simulink model "LQRconlacnguoc"  (R2024b)
settings: Solver=ode45  StartTime=0.0  StopTime=60  FixedStep=0.001  MaxStep=0.01  RelTol=1e-3
values from neighbouring files (symbols this model uses):
  D = [0; 0]    [K_vector_2.m]
libraries: simulink x20, slpidlib x11, slctrl_smc x5, mpclib x1, dspstat3 x1, rllib x1
(part 1 of 3)
settings Model: Creator=DELL  LastModifiedBy=minhh
settings RTWCC: GenCodeOnly=on

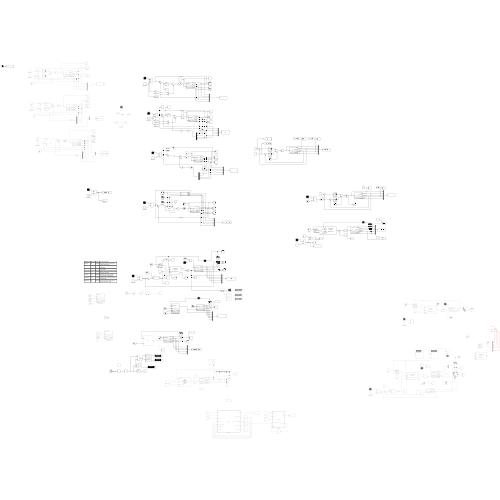
[thumbnail: Simulink's stored preview of the top-level diagram]
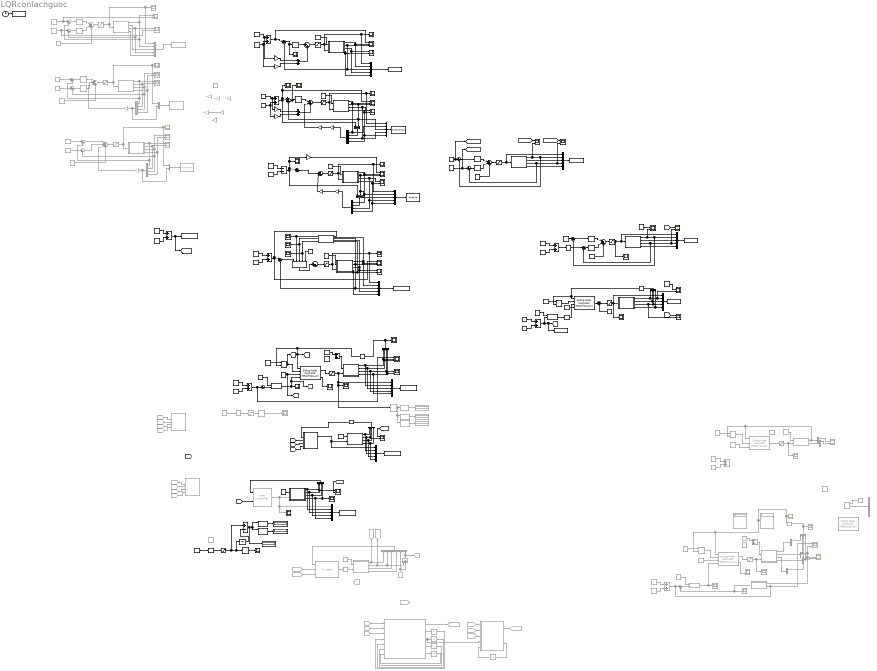
== system LQRconlacnguoc ==
  note: To Improve...
      | Parameter
      | Action
      | The "Physics" Reason
      |
      | Rise Time
      | Eta
      | Increase
      | It increases the force used to "jump" onto the sliding surface.
      |
      | Rise Time
      | C (Slope)
      | Increase
      | It makes the "slide" toward the target much steeper.
      |
      | Settling Time
      | C (Slope)
      | Increase
      | Faster convergence once the system is on the surface.
      |
      | Settling Time
      | Phi
      | Increase
      | Reduces "bouncing" at the target, letting the system rest sooner.
      |
      | S.S. Error
      | Phi
      | Decrease
      | Shrinks the "lazy zone" where the controller stops being aggressive.
      |
      | Smoothness
      | Phi
      | Increase
      | Softens the high-frequency switching (kills chattering).
      |
      | Smoothness
      | Eta
      | Decrease
      | Prevents the system from hitting the sliding surface too violently.
  A : Constant  Commented=on  Value=[0 0 0 0; 0 0 0 1; -4 1 -0.5 0.4; 0.833 -0.833 0.333 -0.333]
  A_1 : Constant  Commented=on  Value=[0, 1; -3, -0.2]
  A_2 : Constant  Commented=on  Value=[0, 0, 0, 0; 0, 0, 0, 1; -4, 1, -0.5, 0.4; 0.833, -0.833, 0.333, -0.333]  VectorParams1D=off
  A_3 : Constant  Value=[0, 0, 0, 0; 0, 0, 0, 1; -4, 1, -0.5, 0.4; 0.833, -0.833, 0.333, -0.333]  VectorParams1D=off
  A_4 : Constant  Value=[0, 1, 0, 0; 29.8310, 0, 0, 0; 0, 0, 0, 1; -0.9392, 0, 0, 0]  VectorParams1D=off
  Add{,2..3,5..7,12..13,16,18} (10 alike) : Sum
  Add1 : Sum  Commented=on
  Add10 : Sum  Commented=on
  Add11 : Sum  Commented=on
  Add14 : Sum  Commented=on  Inputs=-+
  Add15 : Sum  Inputs=+-
  Add4 : Sum  Inputs=+-
  Add8 : Sum  Inputs=--
  Add9 : Sum  Inputs=+-
  Assignment : Assignment  Commented=on  DiagnosticForDimensions=Warning  IndexOptions=Index vector (dialog)  Indices=2  OutputSizes=1
  Assignment1 : Assignment  DiagnosticForDimensions=Warning  IndexOptions=Index vector (dialog)  Indices=2  OutputSizes=1
  Assignment2 : Assignment  DiagnosticForDimensions=Warning  IndexOptions=Index vector (dialog)  Indices=3  OutputSizes=1
  B : Constant  Commented=on  Value=[0; 0.004]
  B1 : Constant  Commented=on  Value=[0; 0; 0.004; 0]
  B2 : Constant  Commented=on  Value=[0; 0.004; 0; 0]
  B3 : Constant  Value=[0; 0.004; 0; 0]
  B4 : Constant  Value=[0; -1.1574; 0; 0.4167]
  Band-Limited White Noise : simulink/Sources/Band-Limited White Noise  Commented=on  Cov=[0.001]  Ts=0.01  seed=[23341]
  Band-Limited White Noise1 : simulink/Sources/Band-Limited White Noise  Commented=on  Cov=[0.001]  Ts=0.01  seed=[23341]
  Band-Limited White Noise{3..5,7,9..11} (7 alike) : simulink/Sources/Band-Limited White Noise  Cov=[200]  Ts=0.01  seed=[23341]
  Band-Limited White Noise12 : simulink/Sources/Band-Limited White Noise  Commented=on  Cov=[200]  Ts=0.01  seed=[23341]
  Band-Limited White Noise13 : simulink/Sources/Band-Limited White Noise  Cov=[0.001]  Ts=0.01  seed=[23341]
  Band-Limited White Noise14 : simulink/Sources/Band-Limited White Noise  Cov=[0.001]  Ts=0.01  seed=[23341]
  Band-Limited White Noise15 : simulink/Sources/Band-Limited White Noise  Cov=[0.001]  Ts=0.01  seed=[23341]
  Band-Limited White Noise2 : simulink/Sources/Band-Limited White Noise  Commented=on  Cov=[0.001]  Ts=0.01  seed=[23341]
  Band-Limited White Noise6 : simulink/Sources/Band-Limited White Noise  Commented=on  Cov=[200]  Ts=0.01  seed=[23341]
  Band-Limited White Noise8 : simulink/Sources/Band-Limited White Noise  Commented=on  Cov=[200]  Ts=0.01  seed=[23341]
  Clock : Clock
      settings: Decimation=100
  Constant : Constant  Commented=on  Value=[0; 0; 0; 0]  VectorParams1D=off
  Constant1 : Constant  Value=[0; 0; 0; 0]  VectorParams1D=off
  Constant2 : Constant  Value=[0; 0; 0; 0]  VectorParams1D=off
  Constant3 : Constant  Value=0
  D_values : Scope
  Demux{,1..5} (6 alike) : Demux  Commented=on  Outputs=2
  Display{,1,5..7} (5 alike) : Display  Commented=on
  Display2 : Display
  Display3 : Display
  Display4 : Display
  Feedforward : Gain  Gain=130  Multiplication=Matrix(K*u)
  Feedforward1 : Gain  Gain=200  Multiplication=Matrix(K*u)
  Feedforward2 : Gain  Gain=300  Multiplication=Matrix(K*u)
  Feedforward3 : Gain  Gain=300  Multiplication=Matrix(K*u)
  From : From  Commented=on  GotoTag=f_x
  From1 : From  Commented=on  GotoTag=x
  From10 : From  Commented=on  GotoTag=x
  From11 : From  Commented=on  GotoTag=g_x
  From12 : From  Commented=on  GotoTag=x_ref
  From15 : From  Commented=on  GotoTag=NN_x2_ref
  From16 : From  Commented=on  GotoTag=NN_Error
  From17 : From  Commented=on  GotoTag=NN_u
  From18 : From  Commented=on  GotoTag=NN_x1
  From19 : From  Commented=on  GotoTag=NN_x2
  From2 : From  Commented=on  GotoTag=g_x
  From20 : From  Commented=on  GotoTag=NN_x2_ref
  From21 : From  Commented=on  GotoTag=NN_x2
  From22 : From  Commented=on  GotoTag=NN_x2_ref
  From23 : From  Commented=on  GotoTag=NN_IsDone
  From24 : From  Commented=on  GotoTag=NN_Reward
  From3 : From  Commented=on  GotoTag=x_ref
  From9 : From  Commented=on  GotoTag=f_x
  Gain1 : Gain  Commented=on  Gain=[-137.7896 -25.9783 -22.3607 -27.5768]  Multiplication=Matrix(K*u)
  Gain10 : Gain  Commented=on  Gain=10000  Multiplication=Matrix(K*u)
  Gain11 : Gain  Commented=on  Gain=[-31.2820 70.3549 95.2844 249.5836]  Multiplication=Matrix(K*u)
  Gain12 : Gain  Commented=on  Gain=[-0.5120 271.0493 500.9119 924.2311]  Multiplication=Matrix(K*u)
  Gain13 : Gain  Gain=-1  Multiplication=Matrix(K*u)
  Gain14 : Gain  Gain="[242.4879  684.9939   85.7051  920.8251]"  Multiplication=Matrix(K*u)
  Gain2 : Gain  Commented=on  Gain=[-137.7896 -25.9783 -22.3607 -27.5768]  Multiplication=Matrix(K*u)
  Gain3 : Gain  Gain="[197.1274  543.9573  131.0655  963.0780]"  Multiplication=Matrix(K*u)
  Gain4 : Gain  Commented=on  Gain=[1.6728 1.0816 0.3095 1.2849]  Multiplication=Matrix(K*u)
  Gain5 : Gain  Commented=on  Gain=[-0.4237 1.7558 1.8822 4.6801]  Multiplication=Matrix(K*u)
  Gain6 : Gain  Multiplication=Matrix(K*u)
  Gain7 : Gain  Gain=.66  Multiplication=Matrix(K*u)
  Gain8 : Gain  Commented=on  Gain=[1.6728 1.0816 0.3095 1.2849]  Multiplication=Matrix(K*u)
  Goto10 : Goto  Commented=on  GotoTag=NN_x2
  Goto5 : Goto  Commented=on  GotoTag=NN_Error
  Goto6 : Goto  Commented=on  GotoTag=NN_u
  Goto7 : Goto  Commented=on  GotoTag=NN_Reward
  Goto8 : Goto  Commented=on  GotoTag=NN_IsDone
  Goto9 : Goto  Commented=on  GotoTag=NN_x1
  I_values : Scope
  IsDone : MATLAB Function  Commented=on  TreatAsAtomicUnit=on
  MPC Controller : mpclib/MPC Controller  Commented=on  SCDEnableBlockLinearizationSpecification=on  mpcobj=mpc1  is_multiple=0  enable_value=0  return_u0=off  updateMPCinCallerWorkspace=on  md_inport=off  mv_inport=off  uref_inport=off  return_cost=off  return_mvseq=off  return_qpstatus=off  return_xseq=off  return_state=off  return_ovseq=off  state_inport=off  umin_inport=off  umax_inport=off  ymin_inport=off  ymax_inport=off  cc_inport=off  ywt_inport=off  uwt_inport=off  duwt_inport=off  rhoeps_inport=off  pm_inport=off  MaximumP=10  HorizonChoice=FixedHorizon  n_ts=0.01  n_p=50  n_mv=1  n_md=0  n_ud=0  n_mo=4  n_uo=0  BlockDataType=double  SampleTimeInherited=off  switch_inport=off
  Manual SMC : Subsystem  Commented=on
  Manual SMC Adaptive : Subsystem
  MatrixMultiply : Product  Commented=on  Multiplication=Matrix(*)
  MatrixMultiply1 : Product  Commented=on  Multiplication=Matrix(*)
  MatrixMultiply2 : Product  Commented=on  Multiplication=Matrix(*)
  MatrixMultiply3 : Product  Multiplication=Matrix(*)
  MatrixMultiply4 : Product  Multiplication=Matrix(*)
  Mean : dspstat3/Mean  Commented=on  run=on  InputProcessing=Columns as channels (frame based)  reset_popup=None  directionMode=Each column  dimension=1  roiEnable=off  roiType=Rectangles  roiPortion=Entire ROI  roiOutput=Individual statistics for each ROI  roiFlag=off  roundingMode=Floor  overflowMode=off  outputDataTypeStr=Inherit: Same as accumulator  outputMin=[]  outputMax=[]  outputLastDataTypeStr=Inherit: Same as accumulator
  MinMax Running Resettable : simulink/Math Operations/MinMax Running Resettable  Function=min  vinit=0.0
  MinMax Running Resettable1 : simulink/Math Operations/MinMax Running Resettable  Function=max  vinit=0.0
  MinMax Running Resettable2 : simulink/Math Operations/MinMax Running Resettable  Commented=on  Function=min  vinit=0.0
  MinMax Running Resettable3 : simulink/Math Operations/MinMax Running Resettable  Commented=on  Function=max  vinit=0.0
  Mux{,1,11,13} (4 alike) : Mux  Commented=on
  Mux{7,9..10,14,16..18,20..22} (10 alike) : Mux  Inputs=5
  Mux{5..6,8,12,15,23} (6 alike) : Mux
  Mux19 : Mux  Commented=on  Inputs=6
  Mux2 : Mux  Commented=on  Inputs=2
  Mux3 : Mux  Commented=on  Inputs=2
  Mux4 : Mux  Commented=on  Inputs=5
  N : Constant  Value=100
  PI : Subsystem  Commented=on
  PID Controller : slpidlib/PID Controller  Commented=on  Controller=PID  Form=Parallel  TimeDomain=Continuous-time  UseExternalTs=off  SampleTime=-1  IntegratorMethod=Forward Euler  FilterMethod=Forward Euler  ControllerParametersSource=internal  P=-40  I=0  UseKiTs=off  D=-8  UseExternalDerivativeSource=off  N=100  UseFilter=on  TunerSelectOption=Transfer Function Based (PID Tuner App)  InitialConditionSource=internal  InitialConditionForIntegrator=0  InitialConditionForFilter=0  DifferentiatorICPrevScaledInput=0  ExternalReset=none  TrackingMode=off  Kt=1  LimitOutput=on  SatLimitsSource=internal  UpperSaturationLimit=1  LowerSaturationLimit=-1  LinearizeAsGain=on  AntiWindupMode=none  Kb=1  LimitIntegrator=off  UpperIntegratorSaturationLimit=inf  LowerIntegratorSaturationLimit=-inf  POutMin=[]  POutMax=[]  IOutMin=[]  IOutMax=[]  DOutMin=[]  DOutMax=[]  NOutMin=[]  NOutMax=[]  SumOutMin=[]  SumOutMax=[]  SaturationOutMin=[]  SaturationOutMax=[]  PParamMin=[]  PParamMax=[]  IParamMin=[]  IParamMax=[]  DParamMin=[]  DParamMax=[]  NParamMin=[]  NParamMax=[]  KbParamMin=[]  KbParamMax=[]  KtParamMin=[]  KtParamMax=[]  KbOutMin=[]  KbOutMax=[]  KtOutMin=[]  KtOutMax=[]  IntegratorOutMin=[]  IntegratorOutMax=[]  FilterOutMin=[]  FilterOutMax=[]  SumI1OutMin=[]  SumI1OutMax=[]  SumI2OutMin=[]  SumI2OutMax=[]  SumI3OutMin=[]  SumI3OutMax=[]  SumI4OutMin=[]  SumI4OutMax=[]  SumDOutMin=[]  SumDOutMax=[]  DifferentiatorOutMin=[]  DifferentiatorOutMax=[]  FilterDiffOutCoefMin=[]  FilterDiffOutCoefMax=[]  ReciprocalOutMin=[]  ReciprocalOutMax=[]  SumDenOutMin=[]  SumDenOutMax=[]  SumNumOutMin=[]  SumNumOutMax=[]  DivideOutMin=[]  DivideOutMax=[]  UdiffTsProdOutMin=[]  UdiffTsProdOutMax=[]  NTsProdOutMin=[]  NTsProdOutMax=[]  UintegralTsProdOutMin=[]  UintegralTsProdOutMax=[]  UngainTsProdOutMin=[]  UngainTsProdOutMax=[]  ClampingZeroOutDataTypeStr=Inherit: Inherit via back propagation  ClampingZeroOutMin=[]  ClampingZeroOutMax=[]  FilterDenConstantOutDataTypeStr=Inherit: Inherit via back propagation  FilterDenConstantOutMin=[]  FilterDenConstantOutMax=[]  PCopyOutDataTypeStr=Inherit: Inherit via back propagation  PCopyOutMin=[]  PCopyOutMax=[]  NCopyOutDataTypeStr=Inherit: Inherit via back propagation  NCopyOutMin=[]  NCopyOutMax=[]  IntegratorContinuousStateAttributes=''  IntegratorStateMustResolveToSignalObject=off  IntegratorRTWStateStorageClass=Auto  FilterContinuousStateAttributes=''  FilterStateMustResolveToSignalObject=off  FilterRTWStateStorageClass=Auto  ParallelPVariant=InternalParameters  IdealPVariant=Disabled  IVariant=InternalParameters  DVariant=InternalParameters  IntegratorVariant=Continuous  SatVariant=Enabled  AWVariant=Passthrough  PCopyVariant=Disabled  TRVariant=Disabled  FdbkBlocksVariant=Forward  IdealPFdbkVariant=Disabled  SatFdbkVariant=Disabled  DerivativeFilterVariant=ContFilter  NVariant=InternalParameters  NCopyVariant=Disabled  FilterICVariant=InternalICsFilter  IntegratorICVariant=InternalICs  ExternalResetVariant=Disabled  TRSumVariant=Passthrough  SumFdbkVariant=Disabled  SumVariant=Sum_PID  TsampFilterVariant=InternalTs  TsampNgainVariant=Passthrough  TsampIntegralVariant=Disabled_SignalSpec  ExternalSaturationOutDataTypeStr=Inherit: Same as second input  DerivativeSourceVariant=ErrorSignal  PreIntVariant=InternalPreInt
  PID Controller1 : slpidlib/PID Controller  Commented=on  Controller=PID  Form=Parallel  TimeDomain=Continuous-time  UseExternalTs=off  SampleTime=-1  IntegratorMethod=Forward Euler  FilterMethod=Forward Euler  ControllerParametersSource=internal  P=-1.25  I=0  UseKiTs=off  D=-3.6  UseExternalDerivativeSource=off  N=100  UseFilter=on  TunerSelectOption=Transfer Function Based (PID Tuner App)  InitialConditionSource=internal  InitialConditionForIntegrator=0  InitialConditionForFilter=0  DifferentiatorICPrevScaledInput=0  ExternalReset=none  TrackingMode=off  Kt=1  LimitOutput=on  SatLimitsSource=internal  UpperSaturationLimit=0.1  LowerSaturationLimit=-0.1  LinearizeAsGain=on  AntiWindupMode=none  Kb=1  LimitIntegrator=off  UpperIntegratorSaturationLimit=inf  LowerIntegratorSaturationLimit=-inf  POutMin=[]  POutMax=[]  IOutMin=[]  IOutMax=[]  DOutMin=[]  DOutMax=[]  NOutMin=[]  NOutMax=[]  SumOutMin=[]  SumOutMax=[]  SaturationOutMin=[]  SaturationOutMax=[]  PParamMin=[]  PParamMax=[]  IParamMin=[]  IParamMax=[]  DParamMin=[]  DParamMax=[]  NParamMin=[]  NParamMax=[]  KbParamMin=[]  KbParamMax=[]  KtParamMin=[]  KtParamMax=[]  KbOutMin=[]  KbOutMax=[]  KtOutMin=[]  KtOutMax=[]  IntegratorOutMin=[]  IntegratorOutMax=[]  FilterOutMin=[]  FilterOutMax=[]  SumI1OutMin=[]  SumI1OutMax=[]  SumI2OutMin=[]  SumI2OutMax=[]  SumI3OutMin=[]  SumI3OutMax=[]  SumI4OutMin=[]  SumI4OutMax=[]  SumDOutMin=[]  SumDOutMax=[]  DifferentiatorOutMin=[]  DifferentiatorOutMax=[]  FilterDiffOutCoefMin=[]  FilterDiffOutCoefMax=[]  ReciprocalOutMin=[]  ReciprocalOutMax=[]  SumDenOutMin=[]  SumDenOutMax=[]  SumNumOutMin=[]  SumNumOutMax=[]  DivideOutMin=[]  DivideOutMax=[]  UdiffTsProdOutMin=[]  UdiffTsProdOutMax=[]  NTsProdOutMin=[]  NTsProdOutMax=[]  UintegralTsProdOutMin=[]  UintegralTsProdOutMax=[]  UngainTsProdOutMin=[]  UngainTsProdOutMax=[]  ClampingZeroOutDataTypeStr=Inherit: Inherit via back propagation  ClampingZeroOutMin=[]  ClampingZeroOutMax=[]  FilterDenConstantOutDataTypeStr=Inherit: Inherit via back propagation  FilterDenConstantOutMin=[]  FilterDenConstantOutMax=[]  PCopyOutDataTypeStr=Inherit: Inherit via back propagation  PCopyOutMin=[]  PCopyOutMax=[]  NCopyOutDataTypeStr=Inherit: Inherit via back propagation  NCopyOutMin=[]  NCopyOutMax=[]  IntegratorContinuousStateAttributes=''  IntegratorStateMustResolveToSignalObject=off  IntegratorRTWStateStorageClass=Auto  FilterContinuousStateAttributes=''  FilterStateMustResolveToSignalObject=off  FilterRTWStateStorageClass=Auto  ParallelPVariant=InternalParameters  IdealPVariant=Disabled  IVariant=InternalParameters  DVariant=InternalParameters  IntegratorVariant=Continuous  SatVariant=Enabled  AWVariant=Passthrough  PCopyVariant=Disabled  TRVariant=Disabled  FdbkBlocksVariant=Forward  IdealPFdbkVariant=Disabled  SatFdbkVariant=Disabled  DerivativeFilterVariant=ContFilter  NVariant=InternalParameters  NCopyVariant=Disabled  FilterICVariant=InternalICsFilter  IntegratorICVariant=InternalICs  ExternalResetVariant=Disabled  TRSumVariant=Passthrough  SumFdbkVariant=Disabled  SumVariant=Sum_PID  TsampFilterVariant=InternalTs  TsampNgainVariant=Passthrough  TsampIntegralVariant=Disabled_SignalSpec  ExternalSaturationOutDataTypeStr=Inherit: Same as second input  DerivativeSourceVariant=ErrorSignal  PreIntVariant=InternalPreInt
  PID Controller2 : slpidlib/PID Controller  Commented=on  Controller=PID  Form=Parallel  TimeDomain=Continuous-time  UseExternalTs=off  SampleTime=-1  IntegratorMethod=Forward Euler  FilterMethod=Forward Euler  ControllerParametersSource=internal  P=1  I=1  UseKiTs=off  D=1  UseExternalDerivativeSource=off  N=100  UseFilter=on  TunerSelectOption=Transfer Function Based (PID Tuner App)  InitialConditionSource=internal  InitialConditionForIntegrator=0  InitialConditionForFilter=0  DifferentiatorICPrevScaledInput=0  ExternalReset=none  TrackingMode=off  Kt=1  LimitOutput=off  SatLimitsSource=internal  UpperSaturationLimit=1  LowerSaturationLimit=-1  LinearizeAsGain=on  AntiWindupMode=none  Kb=1  LimitIntegrator=off  UpperIntegratorSaturationLimit=inf  LowerIntegratorSaturationLimit=-inf  POutMin=[]  POutMax=[]  IOutMin=[]  IOutMax=[]  DOutMin=[]  DOutMax=[]  NOutMin=[]  NOutMax=[]  SumOutMin=[]  SumOutMax=[]  SaturationOutMin=[]  SaturationOutMax=[]  PParamMin=[]  PParamMax=[]  IParamMin=[]  IParamMax=[]  DParamMin=[]  DParamMax=[]  NParamMin=[]  NParamMax=[]  KbParamMin=[]  KbParamMax=[]  KtParamMin=[]  KtParamMax=[]  KbOutMin=[]  KbOutMax=[]  KtOutMin=[]  KtOutMax=[]  IntegratorOutMin=[]  IntegratorOutMax=[]  FilterOutMin=[]  FilterOutMax=[]  SumI1OutMin=[]  SumI1OutMax=[]  SumI2OutMin=[]  SumI2OutMax=[]  SumI3OutMin=[]  SumI3OutMax=[]  SumI4OutMin=[]  SumI4OutMax=[]  SumDOutMin=[]  SumDOutMax=[]  DifferentiatorOutMin=[]  DifferentiatorOutMax=[]  FilterDiffOutCoefMin=[]  FilterDiffOutCoefMax=[]  ReciprocalOutMin=[]  ReciprocalOutMax=[]  SumDenOutMin=[]  SumDenOutMax=[]  SumNumOutMin=[]  SumNumOutMax=[]  DivideOutMin=[]  DivideOutMax=[]  UdiffTsProdOutMin=[]  UdiffTsProdOutMax=[]  NTsProdOutMin=[]  NTsProdOutMax=[]  UintegralTsProdOutMin=[]  UintegralTsProdOutMax=[]  UngainTsProdOutMin=[]  UngainTsProdOutMax=[]  ClampingZeroOutDataTypeStr=Inherit: Inherit via back propagation  ClampingZeroOutMin=[]  ClampingZeroOutMax=[]  FilterDenConstantOutDataTypeStr=Inherit: Inherit via back propagation  FilterDenConstantOutMin=[]  FilterDenConstantOutMax=[]  PCopyOutDataTypeStr=Inherit: Inherit via back propagation  PCopyOutMin=[]  PCopyOutMax=[]  NCopyOutDataTypeStr=Inherit: Inherit via back propagation  NCopyOutMin=[]  NCopyOutMax=[]  IntegratorContinuousStateAttributes=''  IntegratorStateMustResolveToSignalObject=off  IntegratorRTWStateStorageClass=Auto  FilterContinuousStateAttributes=''  FilterStateMustResolveToSignalObject=off  FilterRTWStateStorageClass=Auto  ParallelPVariant=InternalParameters  IdealPVariant=Disabled  IVariant=InternalParameters  DVariant=InternalParameters  IntegratorVariant=Continuous  SatVariant=Disabled  AWVariant=Passthrough  PCopyVariant=Disabled  TRVariant=Disabled  FdbkBlocksVariant=Forward  IdealPFdbkVariant=Disabled  SatFdbkVariant=Disabled  DerivativeFilterVariant=ContFilter  NVariant=InternalParameters  NCopyVariant=Disabled  FilterICVariant=InternalICsFilter  IntegratorICVariant=InternalICs  ExternalResetVariant=Disabled  TRSumVariant=Passthrough  SumFdbkVariant=Disabled  SumVariant=Sum_PID  TsampFilterVariant=InternalTs  TsampNgainVariant=Passthrough  TsampIntegralVariant=Disabled_SignalSpec  ExternalSaturationOutDataTypeStr=Inherit: Same as second input  DerivativeSourceVariant=ErrorSignal  PreIntVariant=InternalPreInt
  PID Controller3 : slpidlib/PID Controller  Commented=on  Controller=PID  Form=Parallel  TimeDomain=Continuous-time  UseExternalTs=off  SampleTime=-1  IntegratorMethod=Forward Euler  FilterMethod=Forward Euler  ControllerParametersSource=internal  P=1.5  I=-7.5  UseKiTs=off  D=5  UseExternalDerivativeSource=off  N=100  UseFilter=on  TunerSelectOption=Transfer Function Based (PID Tuner App)  InitialConditionSource=internal  InitialConditionForIntegrator=0  InitialConditionForFilter=0  DifferentiatorICPrevScaledInput=0  ExternalReset=none  TrackingMode=off  Kt=1  LimitOutput=off  SatLimitsSource=internal  UpperSaturationLimit=0.1  LowerSaturationLimit=-0.1  LinearizeAsGain=on  AntiWindupMode=none  Kb=1  LimitIntegrator=off  UpperIntegratorSaturationLimit=inf  LowerIntegratorSaturationLimit=-inf  POutMin=[]  POutMax=[]  IOutMin=[]  IOutMax=[]  DOutMin=[]  DOutMax=[]  NOutMin=[]  NOutMax=[]  SumOutMin=[]  SumOutMax=[]  SaturationOutMin=[]  SaturationOutMax=[]  PParamMin=[]  PParamMax=[]  IParamMin=[]  IParamMax=[]  DParamMin=[]  DParamMax=[]  NParamMin=[]  NParamMax=[]  KbParamMin=[]  KbParamMax=[]  KtParamMin=[]  KtParamMax=[]  KbOutMin=[]  KbOutMax=[]  KtOutMin=[]  KtOutMax=[]  IntegratorOutMin=[]  IntegratorOutMax=[]  FilterOutMin=[]  FilterOutMax=[]  SumI1OutMin=[]  SumI1OutMax=[]  SumI2OutMin=[]  SumI2OutMax=[]  SumI3OutMin=[]  SumI3OutMax=[]  SumI4OutMin=[]  SumI4OutMax=[]  SumDOutMin=[]  SumDOutMax=[]  DifferentiatorOutMin=[]  DifferentiatorOutMax=[]  FilterDiffOutCoefMin=[]  FilterDiffOutCoefMax=[]  ReciprocalOutMin=[]  ReciprocalOutMax=[]  SumDenOutMin=[]  SumDenOutMax=[]  SumNumOutMin=[]  SumNumOutMax=[]  DivideOutMin=[]  DivideOutMax=[]  UdiffTsProdOutMin=[]  UdiffTsProdOutMax=[]  NTsProdOutMin=[]  NTsProdOutMax=[]  UintegralTsProdOutMin=[]  UintegralTsProdOutMax=[]  UngainTsProdOutMin=[]  UngainTsProdOutMax=[]  ClampingZeroOutDataTypeStr=Inherit: Inherit via back propagation  ClampingZeroOutMin=[]  ClampingZeroOutMax=[]  FilterDenConstantOutDataTypeStr=Inherit: Inherit via back propagation  FilterDenConstantOutMin=[]  FilterDenConstantOutMax=[]  PCopyOutDataTypeStr=Inherit: Inherit via back propagation  PCopyOutMin=[]  PCopyOutMax=[]  NCopyOutDataTypeStr=Inherit: Inherit via back propagation  NCopyOutMin=[]  NCopyOutMax=[]  IntegratorContinuousStateAttributes=''  IntegratorStateMustResolveToSignalObject=off  IntegratorRTWStateStorageClass=Auto  FilterContinuousStateAttributes=''  FilterStateMustResolveToSignalObject=off  FilterRTWStateStorageClass=Auto  ParallelPVariant=InternalParameters  IdealPVariant=Disabled  IVariant=InternalParameters  DVariant=InternalParameters  IntegratorVariant=Continuous  SatVariant=Disabled  AWVariant=Passthrough  PCopyVariant=Disabled  TRVariant=Disabled  FdbkBlocksVariant=Forward  IdealPFdbkVariant=Disabled  SatFdbkVariant=Disabled  DerivativeFilterVariant=ContFilter  NVariant=InternalParameters  NCopyVariant=Disabled  FilterICVariant=InternalICsFilter  IntegratorICVariant=InternalICs  ExternalResetVariant=Disabled  TRSumVariant=Passthrough  SumFdbkVariant=Disabled  SumVariant=Sum_PID  TsampFilterVariant=InternalTs  TsampNgainVariant=Passthrough  TsampIntegralVariant=Disabled_SignalSpec  ExternalSaturationOutDataTypeStr=Inherit: Same as second input  DerivativeSourceVariant=ErrorSignal  PreIntVariant=InternalPreInt
  PID Controller4 : slpidlib/PID Controller  Controller=PID  Form=Parallel  TimeDomain=Continuous-time  UseExternalTs=off  SampleTime=-1  IntegratorMethod=Forward Euler  FilterMethod=Forward Euler  ControllerParametersSource=internal  P=12000  I=1100  UseKiTs=off  D=5000  UseExternalDerivativeSource=off  N=100  UseFilter=on  TunerSelectOption=Transfer Function Based (PID Tuner App)  InitialConditionSource=internal  InitialConditionForIntegrator=0  InitialConditionForFilter=0  DifferentiatorICPrevScaledInput=0  ExternalReset=none  TrackingMode=off  Kt=1  LimitOutput=off  SatLimitsSource=internal  UpperSaturationLimit=1  LowerSaturationLimit=-1  LinearizeAsGain=on  AntiWindupMode=none  Kb=1  LimitIntegrator=off  UpperIntegratorSaturationLimit=inf  LowerIntegratorSaturationLimit=-inf  POutMin=[]  POutMax=[]  IOutMin=[]  IOutMax=[]  DOutMin=[]  DOutMax=[]  NOutMin=[]  NOutMax=[]  SumOutMin=[]  SumOutMax=[]  SaturationOutMin=[]  SaturationOutMax=[]  PParamMin=[]  PParamMax=[]  IParamMin=[]  IParamMax=[]  DParamMin=[]  DParamMax=[]  NParamMin=[]  NParamMax=[]  KbParamMin=[]  KbParamMax=[]  KtParamMin=[]  KtParamMax=[]  KbOutMin=[]  KbOutMax=[]  KtOutMin=[]  KtOutMax=[]  IntegratorOutMin=[]  IntegratorOutMax=[]  FilterOutMin=[]  FilterOutMax=[]  SumI1OutMin=[]  SumI1OutMax=[]  SumI2OutMin=[]  SumI2OutMax=[]  SumI3OutMin=[]  SumI3OutMax=[]  SumI4OutMin=[]  SumI4OutMax=[]  SumDOutMin=[]  SumDOutMax=[]  DifferentiatorOutMin=[]  DifferentiatorOutMax=[]  FilterDiffOutCoefMin=[]  FilterDiffOutCoefMax=[]  ReciprocalOutMin=[]  ReciprocalOutMax=[]  SumDenOutMin=[]  SumDenOutMax=[]  SumNumOutMin=[]  SumNumOutMax=[]  DivideOutMin=[]  DivideOutMax=[]  UdiffTsProdOutMin=[]  UdiffTsProdOutMax=[]  NTsProdOutMin=[]  NTsProdOutMax=[]  UintegralTsProdOutMin=[]  UintegralTsProdOutMax=[]  UngainTsProdOutMin=[]  UngainTsProdOutMax=[]  ClampingZeroOutDataTypeStr=Inherit: Inherit via back propagation  ClampingZeroOutMin=[]  ClampingZeroOutMax=[]  FilterDenConstantOutDataTypeStr=Inherit: Inherit via back propagation  FilterDenConstantOutMin=[]  FilterDenConstantOutMax=[]  PCopyOutDataTypeStr=Inherit: Inherit via back propagation  PCopyOutMin=[]  PCopyOutMax=[]  NCopyOutDataTypeStr=Inherit: Inherit via back propagation  NCopyOutMin=[]  NCopyOutMax=[]  IntegratorContinuousStateAttributes=''  IntegratorStateMustResolveToSignalObject=off  IntegratorRTWStateStorageClass=Auto  FilterContinuousStateAttributes=''  FilterStateMustResolveToSignalObject=off  FilterRTWStateStorageClass=Auto  ParallelPVariant=InternalParameters  IdealPVariant=Disabled  IVariant=InternalParameters  DVariant=InternalParameters  IntegratorVariant=Continuous  SatVariant=Disabled  AWVariant=Passthrough  PCopyVariant=Disabled  TRVariant=Disabled  FdbkBlocksVariant=Forward  IdealPFdbkVariant=Disabled  SatFdbkVariant=Disabled  DerivativeFilterVariant=ContFilter  NVariant=InternalParameters  NCopyVariant=Disabled  FilterICVariant=InternalICsFilter  IntegratorICVariant=InternalICs  ExternalResetVariant=Disabled  TRSumVariant=Passthrough  SumFdbkVariant=Disabled  SumVariant=Sum_PID  TsampFilterVariant=InternalTs  TsampNgainVariant=Passthrough  TsampIntegralVariant=Disabled_SignalSpec  ExternalSaturationOutDataTypeStr=Inherit: Same as second input  DerivativeSourceVariant=ErrorSignal  PreIntVariant=InternalPreInt
  PID Controller5 : slpidlib/PID Controller  Controller=PID  Form=Parallel  TimeDomain=Continuous-time  UseExternalTs=off  SampleTime=-1  IntegratorMethod=Forward Euler  FilterMethod=Forward Euler  ControllerParametersSource=external  P=12000  I=0  UseKiTs=off  D=5000  UseExternalDerivativeSource=off  N=100  UseFilter=on  TunerSelectOption=Transfer Function Based (PID Tuner App)  InitialConditionSource=internal  InitialConditionForIntegrator=0  InitialConditionForFilter=0  DifferentiatorICPrevScaledInput=0  ExternalReset=none  TrackingMode=off  Kt=1  LimitOutput=off  SatLimitsSource=internal  UpperSaturationLimit=1  LowerSaturationLimit=-1  LinearizeAsGain=on  AntiWindupMode=none  Kb=1  LimitIntegrator=off  UpperIntegratorSaturationLimit=inf  LowerIntegratorSaturationLimit=-inf  POutMin=[]  POutMax=[]  IOutMin=[]  IOutMax=[]  DOutMin=[]  DOutMax=[]  NOutMin=[]  NOutMax=[]  SumOutMin=[]  SumOutMax=[]  SaturationOutMin=[]  SaturationOutMax=[]  PParamMin=[]  PParamMax=[]  IParamMin=[]  IParamMax=[]  DParamMin=[]  DParamMax=[]  NParamMin=[]  NParamMax=[]  KbParamMin=[]  KbParamMax=[]  KtParamMin=[]  KtParamMax=[]  KbOutMin=[]  KbOutMax=[]  KtOutMin=[]  KtOutMax=[]  IntegratorOutMin=[]  IntegratorOutMax=[]  FilterOutMin=[]  FilterOutMax=[]  SumI1OutMin=[]  SumI1OutMax=[]  SumI2OutMin=[]  SumI2OutMax=[]  SumI3OutMin=[]  SumI3OutMax=[]  SumI4OutMin=[]  SumI4OutMax=[]  SumDOutMin=[]  SumDOutMax=[]  DifferentiatorOutMin=[]  DifferentiatorOutMax=[]  FilterDiffOutCoefMin=[]  FilterDiffOutCoefMax=[]  ReciprocalOutMin=[]  ReciprocalOutMax=[]  SumDenOutMin=[]  SumDenOutMax=[]  SumNumOutMin=[]  SumNumOutMax=[]  DivideOutMin=[]  DivideOutMax=[]  UdiffTsProdOutMin=[]  UdiffTsProdOutMax=[]  NTsProdOutMin=[]  NTsProdOutMax=[]  UintegralTsProdOutMin=[]  UintegralTsProdOutMax=[]  UngainTsProdOutMin=[]  UngainTsProdOutMax=[]  ClampingZeroOutDataTypeStr=Inherit: Inherit via back propagation  ClampingZeroOutMin=[]  ClampingZeroOutMax=[]  FilterDenConstantOutDataTypeStr=Inherit: Inherit via back propagation  FilterDenConstantOutMin=[]  FilterDenConstantOutMax=[]  PCopyOutDataTypeStr=Inherit: Inherit via back propagation  PCopyOutMin=[]  PCopyOutMax=[]  NCopyOutDataTypeStr=Inherit: Inherit via back propagation  NCopyOutMin=[]  NCopyOutMax=[]  IntegratorContinuousStateAttributes=''  IntegratorStateMustResolveToSignalObject=off  IntegratorRTWStateStorageClass=Auto  FilterContinuousStateAttributes=''  FilterStateMustResolveToSignalObject=off  FilterRTWStateStorageClass=Auto  ParallelPVariant=ExternalParameters  IdealPVariant=Disabled  IVariant=ExternalParameters  DVariant=ExternalParameters  IntegratorVariant=Continuous  SatVariant=Disabled  AWVariant=Passthrough  PCopyVariant=Disabled  TRVariant=Disabled  FdbkBlocksVariant=Forward  IdealPFdbkVariant=Disabled  SatFdbkVariant=Disabled  DerivativeFilterVariant=ContFilter  NVariant=ExternalParameters  NCopyVariant=Disabled  FilterICVariant=InternalICsFilter  IntegratorICVariant=InternalICs  ExternalResetVariant=Disabled  TRSumVariant=Passthrough  SumFdbkVariant=Disabled  SumVariant=Sum_PID  TsampFilterVariant=InternalTs  TsampNgainVariant=Passthrough  TsampIntegralVariant=Disabled_SignalSpec  ExternalSaturationOutDataTypeStr=Inherit: Same as second input  DerivativeSourceVariant=ErrorSignal  PreIntVariant=InternalPreInt
  PID Controller6 : slpidlib/PID Controller  Controller=PID  Form=Parallel  TimeDomain=Continuous-time  UseExternalTs=off  SampleTime=-1  IntegratorMethod=Forward Euler  FilterMethod=Forward Euler  ControllerParametersSource=internal  P=7500  I=1000  UseKiTs=off  D=5000  UseExternalDerivativeSource=off  N=100  UseFilter=on  TunerSelectOption=Transfer Function Based (PID Tuner App)  InitialConditionSource=internal  InitialConditionForIntegrator=0  InitialConditionForFilter=0  DifferentiatorICPrevScaledInput=0  ExternalReset=none  TrackingMode=off  Kt=1  LimitOutput=off  SatLimitsSource=internal  UpperSaturationLimit=1  LowerSaturationLimit=-1  LinearizeAsGain=on  AntiWindupMode=none  Kb=1  LimitIntegrator=off  UpperIntegratorSaturationLimit=inf  LowerIntegratorSaturationLimit=-inf  POutMin=[]  POutMax=[]  IOutMin=[]  IOutMax=[]  DOutMin=[]  DOutMax=[]  NOutMin=[]  NOutMax=[]  SumOutMin=[]  SumOutMax=[]  SaturationOutMin=[]  SaturationOutMax=[]  PParamMin=[]  PParamMax=[]  IParamMin=[]  IParamMax=[]  DParamMin=[]  DParamMax=[]  NParamMin=[]  NParamMax=[]  KbParamMin=[]  KbParamMax=[]  KtParamMin=[]  KtParamMax=[]  KbOutMin=[]  KbOutMax=[]  KtOutMin=[]  KtOutMax=[]  IntegratorOutMin=[]  IntegratorOutMax=[]  FilterOutMin=[]  FilterOutMax=[]  SumI1OutMin=[]  SumI1OutMax=[]  SumI2OutMin=[]  SumI2OutMax=[]  SumI3OutMin=[]  SumI3OutMax=[]  SumI4OutMin=[]  SumI4OutMax=[]  SumDOutMin=[]  SumDOutMax=[]  DifferentiatorOutMin=[]  DifferentiatorOutMax=[]  FilterDiffOutCoefMin=[]  FilterDiffOutCoefMax=[]  ReciprocalOutMin=[]  ReciprocalOutMax=[]  SumDenOutMin=[]  SumDenOutMax=[]  SumNumOutMin=[]  SumNumOutMax=[]  DivideOutMin=[]  DivideOutMax=[]  UdiffTsProdOutMin=[]  UdiffTsProdOutMax=[]  NTsProdOutMin=[]  NTsProdOutMax=[]  UintegralTsProdOutMin=[]  UintegralTsProdOutMax=[]  UngainTsProdOutMin=[]  UngainTsProdOutMax=[]  ClampingZeroOutDataTypeStr=Inherit: Inherit via back propagation  ClampingZeroOutMin=[]  ClampingZeroOutMax=[]  FilterDenConstantOutDataTypeStr=Inherit: Inherit via back propagation  FilterDenConstantOutMin=[]  FilterDenConstantOutMax=[]  PCopyOutDataTypeStr=Inherit: Inherit via back propagation  PCopyOutMin=[]  PCopyOutMax=[]  NCopyOutDataTypeStr=Inherit: Inherit via back propagation  NCopyOutMin=[]  NCopyOutMax=[]  IntegratorContinuousStateAttributes=''  IntegratorStateMustResolveToSignalObject=off  IntegratorRTWStateStorageClass=Auto  FilterContinuousStateAttributes=''  FilterStateMustResolveToSignalObject=off  FilterRTWStateStorageClass=Auto  ParallelPVariant=InternalParameters  IdealPVariant=Disabled  IVariant=InternalParameters  DVariant=InternalParameters  IntegratorVariant=Continuous  SatVariant=Disabled  AWVariant=Passthrough  PCopyVariant=Disabled  TRVariant=Disabled  FdbkBlocksVariant=Forward  IdealPFdbkVariant=Disabled  SatFdbkVariant=Disabled  DerivativeFilterVariant=ContFilter  NVariant=InternalParameters  NCopyVariant=Disabled  FilterICVariant=InternalICsFilter  IntegratorICVariant=InternalICs  ExternalResetVariant=Disabled  TRSumVariant=Passthrough  SumFdbkVariant=Disabled  SumVariant=Sum_PID  TsampFilterVariant=InternalTs  TsampNgainVariant=Passthrough  TsampIntegralVariant=Disabled_SignalSpec  ExternalSaturationOutDataTypeStr=Inherit: Same as second input  DerivativeSourceVariant=ErrorSignal  PreIntVariant=InternalPreInt
  PID_Pos : slpidlib/PID Controller  Controller=PID  Form=Parallel  TimeDomain=Continuous-time  UseExternalTs=off  SampleTime=-1  IntegratorMethod=Forward Euler  FilterMethod=Forward Euler  ControllerParametersSource=internal  P=-1.25  I=0  UseKiTs=off  D=-3.6  UseExternalDerivativeSource=off  N=100  UseFilter=on  TunerSelectOption=Transfer Function Based (PID Tuner App)  InitialConditionSource=internal  InitialConditionForIntegrator=0  InitialConditionForFilter=0  DifferentiatorICPrevScaledInput=0  ExternalReset=none  TrackingMode=off  Kt=1  LimitOutput=on  SatLimitsSource=internal  UpperSaturationLimit=0.1  LowerSaturationLimit=-0.1  LinearizeAsGain=on  AntiWindupMode=none  Kb=1  LimitIntegrator=off  UpperIntegratorSaturationLimit=inf  LowerIntegratorSaturationLimit=-inf  POutMin=[]  POutMax=[]  IOutMin=[]  IOutMax=[]  DOutMin=[]  DOutMax=[]  NOutMin=[]  NOutMax=[]  SumOutMin=[]  SumOutMax=[]  SaturationOutMin=[]  SaturationOutMax=[]  PParamMin=[]  PParamMax=[]  IParamMin=[]  IParamMax=[]  DParamMin=[]  DParamMax=[]  NParamMin=[]  NParamMax=[]  KbParamMin=[]  KbParamMax=[]  KtParamMin=[]  KtParamMax=[]  KbOutMin=[]  KbOutMax=[]  KtOutMin=[]  KtOutMax=[]  IntegratorOutMin=[]  IntegratorOutMax=[]  FilterOutMin=[]  FilterOutMax=[]  SumI1OutMin=[]  SumI1OutMax=[]  SumI2OutMin=[]  SumI2OutMax=[]  SumI3OutMin=[]  SumI3OutMax=[]  SumI4OutMin=[]  SumI4OutMax=[]  SumDOutMin=[]  SumDOutMax=[]  DifferentiatorOutMin=[]  DifferentiatorOutMax=[]  FilterDiffOutCoefMin=[]  FilterDiffOutCoefMax=[]  ReciprocalOutMin=[]  ReciprocalOutMax=[]  SumDenOutMin=[]  SumDenOutMax=[]  SumNumOutMin=[]  SumNumOutMax=[]  DivideOutMin=[]  DivideOutMax=[]  UdiffTsProdOutMin=[]  UdiffTsProdOutMax=[]  NTsProdOutMin=[]  NTsProdOutMax=[]  UintegralTsProdOutMin=[]  UintegralTsProdOutMax=[]  UngainTsProdOutMin=[]  UngainTsProdOutMax=[]  ClampingZeroOutDataTypeStr=Inherit: Inherit via back propagation  ClampingZeroOutMin=[]  ClampingZeroOutMax=[]  FilterDenConstantOutDataTypeStr=Inherit: Inherit via back propagation  FilterDenConstantOutMin=[]  FilterDenConstantOutMax=[]  PCopyOutDataTypeStr=Inherit: Inherit via back propagation  PCopyOutMin=[]  PCopyOutMax=[]  NCopyOutDataTypeStr=Inherit: Inherit via back propagation  NCopyOutMin=[]  NCopyOutMax=[]  IntegratorContinuousStateAttributes=''  IntegratorStateMustResolveToSignalObject=off  IntegratorRTWStateStorageClass=Auto  FilterContinuousStateAttributes=''  FilterStateMustResolveToSignalObject=off  FilterRTWStateStorageClass=Auto  ParallelPVariant=InternalParameters  IdealPVariant=Disabled  IVariant=InternalParameters  DVariant=InternalParameters  IntegratorVariant=Continuous  SatVariant=Enabled  AWVariant=Passthrough  PCopyVariant=Disabled  TRVariant=Disabled  FdbkBlocksVariant=Forward  IdealPFdbkVariant=Disabled  SatFdbkVariant=Disabled  DerivativeFilterVariant=ContFilter  NVariant=InternalParameters  NCopyVariant=Disabled  FilterICVariant=InternalICsFilter  IntegratorICVariant=InternalICs  ExternalResetVariant=Disabled  TRSumVariant=Passthrough  SumFdbkVariant=Disabled  SumVariant=Sum_PID  TsampFilterVariant=InternalTs  TsampNgainVariant=Passthrough  TsampIntegralVariant=Disabled_SignalSpec  ExternalSaturationOutDataTypeStr=Inherit: Same as second input  DerivativeSourceVariant=ErrorSignal  PreIntVariant=InternalPreInt
  PID_Pos1 : slpidlib/PID Controller  Controller=PID  Form=Parallel  TimeDomain=Continuous-time  UseExternalTs=off  SampleTime=-1  IntegratorMethod=Forward Euler  FilterMethod=Forward Euler  ControllerParametersSource=internal  P=-1.25  I=0  UseKiTs=off  D=-3.6  UseExternalDerivativeSource=off  N=100  UseFilter=on  TunerSelectOption=Transfer Function Based (PID Tuner App)  InitialConditionSource=internal  InitialConditionForIntegrator=0  InitialConditionForFilter=0  DifferentiatorICPrevScaledInput=0  ExternalReset=none  TrackingMode=off  Kt=1  LimitOutput=on  SatLimitsSource=internal  UpperSaturationLimit=0.1  LowerSaturationLimit=-0.1  LinearizeAsGain=on  AntiWindupMode=none  Kb=1  LimitIntegrator=off  UpperIntegratorSaturationLimit=inf  LowerIntegratorSaturationLimit=-inf  POutMin=[]  POutMax=[]  IOutMin=[]  IOutMax=[]  DOutMin=[]  DOutMax=[]  NOutMin=[]  NOutMax=[]  SumOutMin=[]  SumOutMax=[]  SaturationOutMin=[]  SaturationOutMax=[]  PParamMin=[]  PParamMax=[]  IParamMin=[]  IParamMax=[]  DParamMin=[]  DParamMax=[]  NParamMin=[]  NParamMax=[]  KbParamMin=[]  KbParamMax=[]  KtParamMin=[]  KtParamMax=[]  KbOutMin=[]  KbOutMax=[]  KtOutMin=[]  KtOutMax=[]  IntegratorOutMin=[]  IntegratorOutMax=[]  FilterOutMin=[]  FilterOutMax=[]  SumI1OutMin=[]  SumI1OutMax=[]  SumI2OutMin=[]  SumI2OutMax=[]  SumI3OutMin=[]  SumI3OutMax=[]  SumI4OutMin=[]  SumI4OutMax=[]  SumDOutMin=[]  SumDOutMax=[]  DifferentiatorOutMin=[]  DifferentiatorOutMax=[]  FilterDiffOutCoefMin=[]  FilterDiffOutCoefMax=[]  ReciprocalOutMin=[]  ReciprocalOutMax=[]  SumDenOutMin=[]  SumDenOutMax=[]  SumNumOutMin=[]  SumNumOutMax=[]  DivideOutMin=[]  DivideOutMax=[]  UdiffTsProdOutMin=[]  UdiffTsProdOutMax=[]  NTsProdOutMin=[]  NTsProdOutMax=[]  UintegralTsProdOutMin=[]  UintegralTsProdOutMax=[]  UngainTsProdOutMin=[]  UngainTsProdOutMax=[]  ClampingZeroOutDataTypeStr=Inherit: Inherit via back propagation  ClampingZeroOutMin=[]  ClampingZeroOutMax=[]  FilterDenConstantOutDataTypeStr=Inherit: Inherit via back propagation  FilterDenConstantOutMin=[]  FilterDenConstantOutMax=[]  PCopyOutDataTypeStr=Inherit: Inherit via back propagation  PCopyOutMin=[]  PCopyOutMax=[]  NCopyOutDataTypeStr=Inherit: Inherit via back propagation  NCopyOutMin=[]  NCopyOutMax=[]  IntegratorContinuousStateAttributes=''  IntegratorStateMustResolveToSignalObject=off  IntegratorRTWStateStorageClass=Auto  FilterContinuousStateAttributes=''  FilterStateMustResolveToSignalObject=off  FilterRTWStateStorageClass=Auto  ParallelPVariant=InternalParameters  IdealPVariant=Disabled  IVariant=InternalParameters  DVariant=InternalParameters  IntegratorVariant=Continuous  SatVariant=Enabled  AWVariant=Passthrough  PCopyVariant=Disabled  TRVariant=Disabled  FdbkBlocksVariant=Forward  IdealPFdbkVariant=Disabled  SatFdbkVariant=Disabled  DerivativeFilterVariant=ContFilter  NVariant=InternalParameters  NCopyVariant=Disabled  FilterICVariant=InternalICsFilter  IntegratorICVariant=InternalICs  ExternalResetVariant=Disabled  TRSumVariant=Passthrough  SumFdbkVariant=Disabled  SumVariant=Sum_PID  TsampFilterVariant=InternalTs  TsampNgainVariant=Passthrough  TsampIntegralVariant=Disabled_SignalSpec  ExternalSaturationOutDataTypeStr=Inherit: Same as second input  DerivativeSourceVariant=ErrorSignal  PreIntVariant=InternalPreInt
  PID_Theta : slpidlib/PID Controller  Controller=PID  Form=Parallel  TimeDomain=Continuous-time  UseExternalTs=off  SampleTime=-1  IntegratorMethod=Forward Euler  FilterMethod=Forward Euler  ControllerParametersSource=internal  P=-40  I=0  UseKiTs=off  D=-8  UseExternalDerivativeSource=off  N=100  UseFilter=on  TunerSelectOption=Transfer Function Based (PID Tuner App)  InitialConditionSource=internal  InitialConditionForIntegrator=0  InitialConditionForFilter=0  DifferentiatorICPrevScaledInput=0  ExternalReset=none  TrackingMode=off  Kt=1  LimitOutput=on  SatLimitsSource=internal  UpperSaturationLimit=1  LowerSaturationLimit=-1  LinearizeAsGain=on  AntiWindupMode=none  Kb=1  LimitIntegrator=off  UpperIntegratorSaturationLimit=inf  LowerIntegratorSaturationLimit=-inf  POutMin=[]  POutMax=[]  IOutMin=[]  IOutMax=[]  DOutMin=[]  DOutMax=[]  NOutMin=[]  NOutMax=[]  SumOutMin=[]  SumOutMax=[]  SaturationOutMin=[]  SaturationOutMax=[]  PParamMin=[]  PParamMax=[]  IParamMin=[]  IParamMax=[]  DParamMin=[]  DParamMax=[]  NParamMin=[]  NParamMax=[]  KbParamMin=[]  KbParamMax=[]  KtParamMin=[]  KtParamMax=[]  KbOutMin=[]  KbOutMax=[]  KtOutMin=[]  KtOutMax=[]  IntegratorOutMin=[]  IntegratorOutMax=[]  FilterOutMin=[]  FilterOutMax=[]  SumI1OutMin=[]  SumI1OutMax=[]  SumI2OutMin=[]  SumI2OutMax=[]  SumI3OutMin=[]  SumI3OutMax=[]  SumI4OutMin=[]  SumI4OutMax=[]  SumDOutMin=[]  SumDOutMax=[]  DifferentiatorOutMin=[]  DifferentiatorOutMax=[]  FilterDiffOutCoefMin=[]  FilterDiffOutCoefMax=[]  ReciprocalOutMin=[]  ReciprocalOutMax=[]  SumDenOutMin=[]  SumDenOutMax=[]  SumNumOutMin=[]  SumNumOutMax=[]  DivideOutMin=[]  DivideOutMax=[]  UdiffTsProdOutMin=[]  UdiffTsProdOutMax=[]  NTsProdOutMin=[]  NTsProdOutMax=[]  UintegralTsProdOutMin=[]  UintegralTsProdOutMax=[]  UngainTsProdOutMin=[]  UngainTsProdOutMax=[]  ClampingZeroOutDataTypeStr=Inherit: Inherit via back propagation  ClampingZeroOutMin=[]  ClampingZeroOutMax=[]  FilterDenConstantOutDataTypeStr=Inherit: Inherit via back propagation  FilterDenConstantOutMin=[]  FilterDenConstantOutMax=[]  PCopyOutDataTypeStr=Inherit: Inherit via back propagation  PCopyOutMin=[]  PCopyOutMax=[]  NCopyOutDataTypeStr=Inherit: Inherit via back propagation  NCopyOutMin=[]  NCopyOutMax=[]  IntegratorContinuousStateAttributes=''  IntegratorStateMustResolveToSignalObject=off  IntegratorRTWStateStorageClass=Auto  FilterContinuousStateAttributes=''  FilterStateMustResolveToSignalObject=off  FilterRTWStateStorageClass=Auto  ParallelPVariant=InternalParameters  IdealPVariant=Disabled  IVariant=InternalParameters  DVariant=InternalParameters  IntegratorVariant=Continuous  SatVariant=Enabled  AWVariant=Passthrough  PCopyVariant=Disabled  TRVariant=Disabled  FdbkBlocksVariant=Forward  IdealPFdbkVariant=Disabled  SatFdbkVariant=Disabled  DerivativeFilterVariant=ContFilter  NVariant=InternalParameters  NCopyVariant=Disabled  FilterICVariant=InternalICsFilter  IntegratorICVariant=InternalICs  ExternalResetVariant=Disabled  TRSumVariant=Passthrough  SumFdbkVariant=Disabled  SumVariant=Sum_PID  TsampFilterVariant=InternalTs  TsampNgainVariant=Passthrough  TsampIntegralVariant=Disabled_SignalSpec  ExternalSaturationOutDataTypeStr=Inherit: Same as second input  DerivativeSourceVariant=ErrorSignal  PreIntVariant=InternalPreInt
  PID_Theta1 : slpidlib/PID Controller  Controller=PID  Form=Parallel  TimeDomain=Continuous-time  UseExternalTs=off  SampleTime=-1  IntegratorMethod=Forward Euler  FilterMethod=Forward Euler  ControllerParametersSource=internal  P=-40  I=0  UseKiTs=off  D=-8  UseExternalDerivativeSource=off  N=100  UseFilter=on  TunerSelectOption=Transfer Function Based (PID Tuner App)  InitialConditionSource=internal  InitialConditionForIntegrator=0  InitialConditionForFilter=0  DifferentiatorICPrevScaledInput=0  ExternalReset=none  TrackingMode=off  Kt=1  LimitOutput=on  SatLimitsSource=internal  UpperSaturationLimit=1  LowerSaturationLimit=-1  LinearizeAsGain=on  AntiWindupMode=none  Kb=1  LimitIntegrator=off  UpperIntegratorSaturationLimit=inf  LowerIntegratorSaturationLimit=-inf  POutMin=[]  POutMax=[]  IOutMin=[]  IOutMax=[]  DOutMin=[]  DOutMax=[]  NOutMin=[]  NOutMax=[]  SumOutMin=[]  SumOutMax=[]  SaturationOutMin=[]  SaturationOutMax=[]  PParamMin=[]  PParamMax=[]  IParamMin=[]  IParamMax=[]  DParamMin=[]  DParamMax=[]  NParamMin=[]  NParamMax=[]  KbParamMin=[]  KbParamMax=[]  KtParamMin=[]  KtParamMax=[]  KbOutMin=[]  KbOutMax=[]  KtOutMin=[]  KtOutMax=[]  IntegratorOutMin=[]  IntegratorOutMax=[]  FilterOutMin=[]  FilterOutMax=[]  SumI1OutMin=[]  SumI1OutMax=[]  SumI2OutMin=[]  SumI2OutMax=[]  SumI3OutMin=[]  SumI3OutMax=[]  SumI4OutMin=[]  SumI4OutMax=[]  SumDOutMin=[]  SumDOutMax=[]  DifferentiatorOutMin=[]  DifferentiatorOutMax=[]  FilterDiffOutCoefMin=[]  FilterDiffOutCoefMax=[]  ReciprocalOutMin=[]  ReciprocalOutMax=[]  SumDenOutMin=[]  SumDenOutMax=[]  SumNumOutMin=[]  SumNumOutMax=[]  DivideOutMin=[]  DivideOutMax=[]  UdiffTsProdOutMin=[]  UdiffTsProdOutMax=[]  NTsProdOutMin=[]  NTsProdOutMax=[]  UintegralTsProdOutMin=[]  UintegralTsProdOutMax=[]  UngainTsProdOutMin=[]  UngainTsProdOutMax=[]  ClampingZeroOutDataTypeStr=Inherit: Inherit via back propagation  ClampingZeroOutMin=[]  ClampingZeroOutMax=[]  FilterDenConstantOutDataTypeStr=Inherit: Inherit via back propagation  FilterDenConstantOutMin=[]  FilterDenConstantOutMax=[]  PCopyOutDataTypeStr=Inherit: Inherit via back propagation  PCopyOutMin=[]  PCopyOutMax=[]  NCopyOutDataTypeStr=Inherit: Inherit via back propagation  NCopyOutMin=[]  NCopyOutMax=[]  IntegratorContinuousStateAttributes=''  IntegratorStateMustResolveToSignalObject=off  IntegratorRTWStateStorageClass=Auto  FilterContinuousStateAttributes=''  FilterStateMustResolveToSignalObject=off  FilterRTWStateStorageClass=Auto  ParallelPVariant=InternalParameters  IdealPVariant=Disabled  IVariant=InternalParameters  DVariant=InternalParameters  IntegratorVariant=Continuous  SatVariant=Enabled  AWVariant=Passthrough  PCopyVariant=Disabled  TRVariant=Disabled  FdbkBlocksVariant=Forward  IdealPFdbkVariant=Disabled  SatFdbkVariant=Disabled  DerivativeFilterVariant=ContFilter  NVariant=InternalParameters  NCopyVariant=Disabled  FilterICVariant=InternalICsFilter  IntegratorICVariant=InternalICs  ExternalResetVariant=Disabled  TRSumVariant=Passthrough  SumFdbkVariant=Disabled  SumVariant=Sum_PID  TsampFilterVariant=InternalTs  TsampNgainVariant=Passthrough  TsampIntegralVariant=Disabled_SignalSpec  ExternalSaturationOutDataTypeStr=Inherit: Same as second input  DerivativeSourceVariant=ErrorSignal  PreIntVariant=InternalPreInt
  P_values : Scope
  Pos_H : Scope  NumInputPorts=3
  Pos_LQR : Scope  NumInputPorts=3
  Pos_PID : Scope  NumInputPorts=3
  Pos_PID1 : Scope  NumInputPorts=3
  Pulse Generator{,2..4,10..12,14} (8 alike) : DiscretePulseGenerator  PulseType=Time based  Amplitude=0.3  Period=100  PulseWidth=20  PhaseDelay=20
  Pulse Generator1 : DiscretePulseGenerator  Commented=on  PulseType=Time based  Amplitude=5  Period=10  PulseWidth=50
  Pulse Generator5 : DiscretePulseGenerator  Commented=on  PulseType=Time based  Amplitude=0.3  Period=100  PulseWidth=20  PhaseDelay=20
  Pulse Generator6 : DiscretePulseGenerator  Commented=on  PulseType=Time based  Amplitude=500  Period=100  PulseWidth=.1
  Pulse Generator7 : DiscretePulseGenerator  PulseType=Time based  Amplitude=500  Period=100  PulseWidth=.1
  Pulse Generator8 : DiscretePulseGenerator  Commented=on  PulseType=Time based  Amplitude=500  Period=100  PulseWidth=.1
  Pulse Generator9 : DiscretePulseGenerator  Commented=on  PulseType=Time based  Amplitude=0.3  Period=100  PulseWidth=20  PhaseDelay=20
  RL Agent : rllib/RL Agent  Commented=on  Agent=agentObj  ExternalActionAsInput=off  ProvideLastAction=off  ProvideCumRwd=off  TreatAsDirectFeedthrough=on  UseStrictObservationDataTypes=off
  Rate Limiter : RateLimiter  Commented=on  RisingSlewLimit=25000  FallingSlewLimit=-25000  SampleTimeMode=inherited
  Rate Limiter1 : RateLimiter  Commented=on  RisingSlewLimit=0.1  FallingSlewLimit=-0.1  SampleTimeMode=inherited
  Rate Limiter2 : RateLimiter  RisingSlewLimit=0.15  FallingSlewLimit=-0.15  SampleTimeMode=inherited
  Rate Limiter3 : RateLimiter  RisingSlewLimit=0.1  FallingSlewLimit=-0.1  SampleTimeMode=inherited
  Rate Limiter4 : RateLimiter  Commented=on  RisingSlewLimit=0.1  FallingSlewLimit=-0.1  SampleTimeMode=inherited
  Rate Limiter5 : RateLimiter  RisingSlewLimit=0.15  FallingSlewLimit=-0.15  SampleTimeMode=inherited
  Rate Transition : RateTransition  OutPortSampleTime=0.01
  Rate Transition1 : RateTransition  Commented=on  OutPortSampleTime=0.01
  Rate Transition2 : RateTransition  Commented=on  OutPortSampleTime=0.01
  Ref 1 : Constant  Commented=on  Value=0
  Ref 2 : Constant  Commented=on  Value=0
  Ref Theta : Constant  Commented=on  Value=0
  Ref Theta{1..3,5..6,8,11,14} (8 alike) : Constant  Value=.1
  Ref Theta10 : Constant  Value=0
  Ref Theta4 : Constant  Commented=on  Value=.1
  Ref Theta7 : Constant  Commented=on  Value=.1
  Ref Theta9 : Constant  Value=0
  Ref position : Constant  Commented=on  Value=0.1
  Ref position1 : Constant  Commented=on  Value=0.1
  Ref position2 : Constant  Commented=on  Value=0.1
  Ref position3 : Constant  Value=0.1
  Reshape : Reshape  Commented=on  OutputDimensionality=Column vector (2-D)
  Reshape1 : Reshape  OutputDimensionality=Column vector (2-D)
  Reshape2 : Reshape  OutputDimensionality=Column vector (2-D)
  Reshape3 : Reshape  OutputDimensionality=Column vector (2-D)
  Reward : MATLAB Function  Commented=on  TreatAsAtomicUnit=on
  STW SMC : Subsystem  Commented=on
  Sat_3500 : Saturate  UpperLimit=3500  LowerLimit=-3500
  Saturation : Saturate  Commented=on  UpperLimit=1  LowerLimit=-1
  Saturation1 : Saturate  Commented=on  UpperLimit=1  LowerLimit=-1
  Saturation10 : Saturate  UpperLimit=1  LowerLimit=-1
  Saturation11 : Saturate  Commented=on  LowerLimit=-0.2
  Saturation12 : Saturate  UpperLimit=1  LowerLimit=-1
  Saturation13 : Saturate  UpperLimit=1  LowerLimit=-1
  Saturation2 : Saturate  Commented=on  UpperLimit=1  LowerLimit=-1
  Saturation3 : Saturate  Commented=on  UpperLimit=3500  LowerLimit=-3500
  Saturation{4..6,8} (4 alike) : Saturate  UpperLimit=3500  LowerLimit=-3500
  Saturation7 : Saturate  Commented=on  UpperLimit=3500  LowerLimit=-3500
  Saturation9 : Saturate  LowerLimit=-0.2
  Scope{,1..2,5,17,19..21,23..24,30,33} (12 alike) : Scope
  Scope10 : Scope  Commented=on  NumInputPorts=2
  Scope{7,9,11..12,14..15,26} (7 alike) : Scope  Commented=on
  Scope13 : Scope  Commented=on  NumInputPorts=2
  Scope16 : Scope  NumInputPorts=3
  Scope{3..4,18,25,27..29,31..32} (9 alike) : Scope  NumInputPorts=2
  Scope22 : Scope  NumInputPorts=3
  Scope6 : Scope  Commented=on  NumInputPorts=2
  Scope8 : Scope  Commented=on  NumInputPorts=3
  Sliding Mode Controller (Reaching Law) : slctrl_smc/Sliding Mode Controller (Reaching Law)  Commented=on  TaskMode=Regulation Mode  SlidingMatrix=[1;1]  EnableTrackingDerivative=off  EnableSwitchingFunction=off  ReachingLaw=Constant Rate  ReachingRate=1  ControlGain=0.01  PowerRate=0.01  BoundaryLayer=Saturation  ZeroCross=off  Phi=0.01
  Sliding Mode Controller (Reaching Law)1 : slctrl_smc/Sliding Mode Controller (Reaching Law)  Commented=on  TaskMode=Tracking Mode  SlidingMatrix=[0;10;0;1]  EnableTrackingDerivative=off  EnableSwitchingFunction=off  ReachingLaw=Constant Rate  ReachingRate=1  ControlGain=0.01  PowerRate=0.01  BoundaryLayer=Sign  ZeroCross=off  Phi=0.01
  Sliding Mode Controller (Reaching Law)2 : slctrl_smc/Sliding Mode Controller (Reaching Law)  Commented=on  TaskMode=Tracking Mode  SlidingMatrix=[.1; 3; .1; 4]  EnableTrackingDerivative=off  EnableSwitchingFunction=on  ReachingLaw=Exponential  ReachingRate=1.2  ControlGain=1.5  PowerRate=1  BoundaryLayer=Hyperbolic Tangent  ZeroCross=off  Phi=.5
  Sliding Mode Controller (Reaching Law)3 : slctrl_smc/Sliding Mode Controller (Reaching Law)  TaskMode=Tracking Mode  SlidingMatrix=[0; 8; 0; 4]  EnableTrackingDerivative=off  EnableSwitchingFunction=on  ReachingLaw=Exponential  ReachingRate=20  ControlGain=10  PowerRate=1  BoundaryLayer=Hyperbolic Tangent  ZeroCross=off  Phi=0.0274
  Sliding Mode Controller (Reaching Law)4 : slctrl_smc/Sliding Mode Controller (Reaching Law)  TaskMode=Tracking Mode  SlidingMatrix=[-654.4437; -148.1602; -100; -117.5960]  EnableTrackingDerivative=off  EnableSwitchingFunction=off  ReachingLaw=Exponential  ReachingRate=100  ControlGain=10  PowerRate=1  BoundaryLayer=Hyperbolic Tangent  ZeroCross=off  Phi=1
  Subsystem : Subsystem
  Subsystem1 : Subsystem  Commented=on
  Subsystem10 : Subsystem
  Subsystem11 : Subsystem
  Subsystem12 : Subsystem
  Subsystem13 : Subsystem  Commented=on
  Subsystem14 : Subsystem
  Subsystem15 : Subsystem
  Subsystem16 : Subsystem
  Subsystem2 : Subsystem  Commented=on
  Subsystem3 : Subsystem  Commented=on
  Subsystem4 : Subsystem
  Subsystem5 : Subsystem
  Subsystem6 : Subsystem
  Subsystem7 : Subsystem
  Subsystem8 : Subsystem  Commented=on
  Subsystem9 : Subsystem  Commented=on
  Sum{,1,3..4,6..7} (6 alike) : Sum  Commented=on  Inputs=|+-
  Sum{10..11,18,25} (4 alike) : Sum  Inputs=|++
  Sum12 : Sum  Inputs=|+++--
  Sum13 : Sum  Inputs=|+--
  Sum14 : Sum  Inputs=|+-+
  Sum15 : Sum  Inputs=|+--
  Sum16 : Sum  Commented=on  Inputs=|++
  Sum17 : Sum  Inputs=|-+-+
  Sum{19..20,22..23} (4 alike) : Sum  Inputs=|+-
  Sum2 : Sum  Commented=on  Inputs=|+++
  Sum21 : Sum  Inputs=|+++
  Sum24 : Sum  Inputs=|+++
  Sum5 : Sum  Commented=on  Inputs=|++-+
  Sum8 : Sum  Commented=on  Inputs=|++-+
  Sum9 : Sum  Inputs=|+--
  To Workspace : ToWorkspace  VariableName=t  SaveFormat=Timeseries  SampleTime=-1
  To Workspace1 : ToWorkspace  Commented=on  VariableName=ip_pid_lqr_dist  SampleTime=0.1
  To Workspace10 : ToWorkspace  VariableName=x2_ref  SampleTime=0.1
  To Workspace11 : ToWorkspace  VariableName=cmsd_mpc  SampleTime=0.1
  To Workspace12 : ToWorkspace  VariableName=IP_PID  SaveFormat=Timeseries  SampleTime=-1
  To Workspace13 : ToWorkspace  VariableName=IP_dual_PID  SaveFormat=Timeseries  SampleTime=-1
  To Workspace14 : ToWorkspace  VariableName=ip_x_ref  SaveFormat=Timeseries  SampleTime=-1
  To Workspace15 : ToWorkspace  VariableName=IP_SMC  SaveFormat=Timeseries  SampleTime=-1
  To Workspace2 : ToWorkspace  Commented=on  VariableName=ip_lqr_only  SampleTime=0.1
  To Workspace3 : ToWorkspace  Commented=on  VariableName=ip_pid_only  SampleTime=0.1
  To Workspace4 : ToWorkspace  VariableName=cmsd_pid_lqr  SampleTime=0.1
  To Workspace5 : ToWorkspace  VariableName=cmsd_lqr  SampleTime=0.1
  To Workspace6 : ToWorkspace  VariableName=cmsd_pid  SampleTime=0.1
  To Workspace7 : ToWorkspace  VariableName=cmsd_adaptive_pid  SampleTime=0.1
  To Workspace8 : ToWorkspace  VariableName=cmsd_smc  SampleTime=0.1
  To Workspace9 : ToWorkspace  VariableName=cmsd_adaptive_smc  SampleTime=0.1
  Uniform Random Number : UniformRandomNumber  Minimum=-0.2  Maximum=0.5  Seed=12311  SampleTime=3
  Uniform Random Number2 : UniformRandomNumber  Commented=on  Minimum=-0.2  Maximum=0.5  Seed=12345  SampleTime=3
  Unit Delay{,1..4} (5 alike) : UnitDelay  Commented=on  SampleTime=0.01  HasFrameUpgradeWarning=on
  Unit Delay5 : UnitDelay  SampleTime=3  HasFrameUpgradeWarning=on
  V_H : Scope  NumInputPorts=2
  V_LQR : Scope  NumInputPorts=2
  V_PID : Scope  NumInputPorts=2
  V_PID1 : Scope  NumInputPorts=2
  Zero : Constant  Value=0  OutDataTypeStr=Inherit: Inherit via back propagation
  pos : Scope  Commented=on  NumInputPorts=2
  pos1 : Scope  Commented=on  NumInputPorts=2
  pos2 : Scope  Commented=on  NumInputPorts=2
  theta : Scope  Commented=on  NumInputPorts=2
  theta1 : Scope  Commented=on  NumInputPorts=2
  theta2 : Scope  Commented=on  NumInputPorts=2
  u : Scope  Commented=on
  u1 : Scope  Commented=on
  u2 : Scope  Commented=on
  u{3..6} (4 alike) : Scope
  wires:
  Sum/1 -> PID Controller/1
  Sum1/1 -> PID Controller1/1
  Ref position/1 -> pos/2, Sum1/1
  Ref Theta/1 -> theta/2, Sum/1
  Clock/1 -> To Workspace/1
  Subsystem3/1(góc) -> Sum/2, Mux4/2, theta/1  "Theta"
  Subsystem3/3(vị trí) -> Mux4/4, Sum1/2, pos/1  "Position"
  Sum2/1 -> Saturation/1
  Band-Limited White Noise/1 -> Sum2/3
  PID Controller/1 -> Sum2/1
  PID Controller1/1 -> Sum2/2
  Sum4/1 -> PID Controller3/1
  PID Controller3/1 -> Sum5/2
  Ref 1/1 -> Sum3/1
  Subsystem1/3(vị trí) -> pos1/1, Mux/3, Sum4/2  "x"
  Ref position1/1 -> Sum4/1
  Subsystem1/1(góc) -> Mux/1, Sum3/2, theta1/1  "Theta"
  Sum5/1 -> Saturation1/1
  PID Controller2/1 -> Sum5/1
  Sum3/1 -> PID Controller2/1
  Mux/1 -> Mux2/2, Gain1/1
  Subsystem1/2(góc dot) -> theta1/2, Mux/2  "Thetha dot"
  Subsystem1/4(vị trí dot) -> pos1/2, Mux/4  "x dot"
  Gain1/1 -> Sum5/3
  Band-Limited White Noise1/1 -> Sum5/4
  Saturation1/1 -> Subsystem1/1(u), Mux2/1, u1/1
  Mux2/1 -> To Workspace1/1
  Subsystem2/3(vị trí) -> pos2/1, Mux1/3, Sum7/2  "x"
  Sum7/1 -> Sum8/2
  Mux3/1 -> To Workspace2/1
  Saturation2/1 -> Subsystem2/1(u), Mux3/1, u2/1
  Sum8/1 -> Saturation2/1
  Ref 2/1 -> Sum6/1
  Subsystem2/2(góc dot) -> theta2/2, Mux1/2  "Thetha dot"
  Sum6/1 -> Sum8/1
  Subsystem2/4(vị trí dot) -> pos2/2, Mux1/4  "x dot"
  Ref position2/1 -> Sum7/1
  Gain2/1 -> Sum8/3
  Band-Limited White Noise2/1 -> Sum8/4
  Subsystem2/1(góc) -> Mux1/1, Sum6/2, theta2/1  "Theta"
  Mux1/1 -> Mux3/2, Gain2/1
  Subsystem3/2(góc dot) -> Mux4/3  "Thetha dot"
  Subsystem3/4(vị trí dot) -> Mux4/5  "x dot"
  Mux4/1 -> To Workspace3/1
  Saturation/1 -> Subsystem3/1(u), Mux4/1, u/1
  Gain3/1 -> Gain6/1
  Subsystem4/4(Vel_2) -> Mux7/5, Mux6/4, V_LQR/2  "v2"
  Sum12/1 -> Scope/1, PID Controller6/1
  Subsystem6/2(Pos_2) -> Pos_PID/3, Sum9/3, Mux9/3  "x2"
  Subsystem5/1(Pos_1) -> Mux17/2, Mux5/1, Pos_H/2  "x1"
  Subsystem4/2(Pos_2) -> Pos_LQR/3, Mux7/3, Add9/2  "x2"
  Subsystem5/2(Pos_2) -> Pos_H/3, Mux17/3, Add4/2, Sum12/5  "x2"
  Sum9/1 -> Scope1/1, PID Controller4/1
  Subsystem4/3(Vel_1) -> V_LQR/1, Mux6/3, Mux7/4  "v1"
  Subsystem6/1(Pos_1) -> Mux9/2, Pos_PID/2  "x1"
  Mux6/1 -> Gain14/1
  Subsystem5/4(Vel_2) -> V_H/2, Mux17/5, Mux5/4  "v2"
  Mux5/1 -> Gain3/1
  Subsystem6/3(Vel_1) -> Mux9/4, V_PID/1  "v1"
  PID Controller6/1 -> Sum14/1
  Add8/1 -> Add9/1, Scope5/1, Gain13/1, Sum15/1  "Reference"
  Subsystem6/4(Vel_2) -> V_PID/2, Mux9/5  "v2"
  Mux9/1 -> To Workspace6/1
  Gain14/1 -> Gain7/1
  Subsystem5/3(Vel_1) -> V_H/1, Mux17/4, Mux5/3  "v1"
  Subsystem4/1(Pos_1) -> Mux6/1, Mux7/2, Pos_LQR/2  "x1"
  PID Controller4/1 -> Sum11/1
  Add5/1 -> Pos_PID/1, Sum9/1  "Reference"
  Sum17/1 -> Saturation5/1
  Saturation5/1 -> Subsystem4/2(u (N)), Mux7/1, u5/1
  Sum14/1 -> Sat_3500/1
  Sat_3500/1 -> Subsystem5/2(u (N)), Mux17/1, u4/1
  Sum11/1 -> Saturation4/1
  Saturation4/1 -> Subsystem6/2(u), Mux9/1, u3/1
  Subsystem7/4(Vel_2) -> Subsystem/5(v2), V_PID1/2, Mux10/5  "v2"
  Sum13/1 -> PID Controller5/1
  Mux10/1 -> To Workspace7/1
  Saturation6/1 -> Subsystem7/2(u (N)), Mux10/1, u6/1
  Subsystem7/3(Vel_1) -> Subsystem/4(v1), Mux10/4, V_PID1/1  "v1"
  Subsystem7/2(Pos_2) -> Sum13/3, Mux10/3, Pos_PID1/3, Subsystem/3(x2)  "x2"
  PID Controller5/1 -> Sum10/1
  Subsystem7/1(Pos_1) -> Mux10/2, Pos_PID1/2, Subsystem/2(x1)  "x1"
  Sum10/1 -> Saturation6/1
  Subsystem/3(k_D) -> D_values/1, PID Controller5/4
  Subsystem/2(k_I) -> PID Controller5/3, I_values/1
  Subsystem/1(k_P) -> P_values/1, PID Controller5/2
  N/1 -> PID Controller5/5
  Gain4/1 -> Gain10/1
  Band-Limited White Noise4/1 -> Subsystem6/1(disturbance)
  Band-Limited White Noise3/1 -> Subsystem5/1(disturbance)
  Add/1 -> Add4/1, Pos_H/1, Scope2/1, Sum12/2  "Reference"
  Add4/1 -> Mux5/2
  Pulse Generator/1 -> Feedforward/1, Add/1
  Pulse Generator2/1 -> Feedforward1/1, Add5/1
  Ref Theta5/1 -> Feedforward3/1, Add5/2
  Ref Theta2/1 -> Feedforward2/1, Add/2
  Add6/1 -> Sum14/3
  Feedforward2/1 -> Add6/2
  Feedforward/1 -> Add6/1
  Feedforward3/1 -> Add7/2
  Feedforward1/1 -> Add7/1
  Add7/1 -> Sum11/2
  Pulse Generator3/1 -> Add8/1
  Ref Theta6/1 -> Add8/2
  Gain6/1 -> Sum14/2
  Gain7/1 -> Sum17/3
  Sum15/1 -> Sum17/2
  Add9/1 -> Mux6/2
  Pulse Generator4/1 -> Add2/1
  Ref Theta3/1 -> Add2/2
  Add2/1 -> Pos_PID1/1, Subsystem/1(x_ref), Sum13/1  "Reference"
  Band-Limited White Noise5/1 -> Subsystem4/1(disturbance)
  Band-Limited White Noise7/1 -> Subsystem7/1(disturbance)
  Ref Theta7/1 -> Add1/2
  Pulse Generator5/1 -> Add1/1
  Sliding Mode Controller (Reaching Law)/1 -> Saturation3/1
  Saturation3/1 -> Scope7/1, Subsystem9/2(u)
  Subsystem9/1(x) -> Sliding Mode Controller (Reaching Law)/1, MatrixMultiply1/2, Demux/1  "pos"
  Gain13/1 -> Pos_LQR/1
  B/1 -> Sliding Mode Controller (Reaching Law)/3
  A/1 -> MatrixMultiply/1
  ? -> Mux11/1  "x1"
  ? -> Mux11/2  "x2"
  ? -> Mux11/4  "v2"
  Mux11/1 -> MatrixMultiply/2
  ? -> Mux11/3  "v1"
  MatrixMultiply1/1 -> Sliding Mode Controller (Reaching Law)/2
  A_1/1 -> MatrixMultiply1/1
  Pulse Generator6/1 -> Subsystem9/1(disturbance)
  Subsystem9/2(v) -> Demux1/1  "vel"
  Demux/1 -> Scope6/1  "pos"
  Demux1/1 -> Scope6/2  "vel"
  Demux3/1 -> Scope8/3, Mux13/4  "vel"
  B2/1 -> Sliding Mode Controller (Reaching Law)2/3
  Saturation7/1 -> Subsystem8/2(u (N)), Scope9/1
  Sliding Mode Controller (Reaching Law)2/1 -> Saturation7/1
  A_2/1 -> MatrixMultiply2/1
  MatrixMultiply2/1 -> Sliding Mode Controller (Reaching Law)2/2
  Demux2/1 -> Scope10/2, PI/1(Actual Position), Scope8/2, Mux13/2  "pos"
  Subsystem8/2(Pos_2) -> Demux2/1  "x2"
  Subsystem8/4(Vel_2) -> Demux3/1  "v2"
  Pulse Generator9/1 -> Add11/1
  Ref Theta4/1 -> Add11/2
  Constant/1 -> Assignment/1
  Assignment/1 -> Sliding Mode Controller (Reaching Law)2/4, Scope11/1  "Reference"
  Add11/1 -> PI/2(Reference), Scope10/1, Sum16/1  "Reference"
  Sum16/1 -> Assignment/2
  PI/1(Out) -> Sum16/2, Scope12/1
  Sliding Mode Controller (Reaching Law)2/2 -> Scope13/2
  Band-Limited White Noise8/1 -> Add10/1
  Add10/1 -> Subsystem8/1(disturbance)
  Demux4/1 -> Mux13/1
  Subsystem8/3(Vel_1) -> Demux5/1  "v1"
  Demux5/1 -> Mux13/3
  Mux13/1 -> Reshape/1, Scope14/1
  Reshape/1 -> Sliding Mode Controller (Reaching Law)2/1, MatrixMultiply2/2, Display1/1, Scope15/1
  Subsystem8/1(Pos_1) -> Demux4/1  "x1"
  Subsystem10/3(Vel_1) -> Mux14/4, Scope22/2, Mux12/3  "v1"
  Add12/1 -> Scope16/1, Sum18/1  "Reference"
  Sliding Mode Controller (Reaching Law)3/1 -> Saturation8/1
  Mux12/1 -> Scope20/1, Reshape1/1
  MatrixMultiply3/1 -> [f_x], Sliding Mode Controller (Reaching Law)3/2
  Add3/1 -> Subsystem10/1(disturbance)
  B3/1 -> [g_x], Sliding Mode Controller (Reaching Law)3/3
  Pulse Generator10/1 -> Add12/1
  Subsystem10/1(Pos_1) -> Mux14/2, Scope16/2, Mux12/1  "x1"
  A_3/1 -> MatrixMultiply3/1
  Assignment1/1 -> [x_ref], Sliding Mode Controller (Reaching Law)3/4, Scope17/1  "Reference"
  Sliding Mode Controller (Reaching Law)3/2 -> Scope19/1
  Saturation8/1 -> Subsystem10/2(u (N)), Rate Transition1/1, Scope23/1, Mux14/1
  Ref Theta1/1 -> Add12/2
  Constant1/1 -> Assignment1/1
  Subsystem10/4(Vel_2) -> Scope22/3, Mux12/4, Mux14/5  "v2"
  Reshape1/1 -> MatrixMultiply3/2, [x], Sliding Mode Controller (Reaching Law)3/1
  Subsystem10/2(Pos_2) -> Mux14/3, Scope16/3, Mux12/2  "x2"
  Band-Limited White Noise9/1 -> Add3/1
  Mux14/1 -> To Workspace8/1
  From/1 -> Manual SMC/3(f(x))
  From1/1 -> Manual SMC/2(x)
  From2/1 -> Manual SMC/4(g(x))
  From3/1 -> Manual SMC/5(x_ref)
  [x_ref] -> Manual SMC Adaptive/5(x_ref)
  [f_x] -> Manual SMC Adaptive/3(f(x))
  [g_x] -> Manual SMC Adaptive/4(g(x))
  Band-Limited White Noise10/1 -> Subsystem11/1(disturbance)
  Manual SMC Adaptive/1(u) -> Mux16/1, Subsystem11/2(u (N))
  Subsystem11/2(Pos_2) -> Mux16/3, Scope18/2, Mux15/2  "x2"
  Mux15/1 -> Reshape2/1
  Subsystem11/1(Pos_1) -> Mux16/2, Mux15/1  "x1"
  Subsystem11/3(Vel_1) -> Mux16/4, Mux15/3  "v1"
  Subsystem11/4(Vel_2) -> Mux16/5, Mux15/4  "v2"
  Reshape2/1 -> Manual SMC Adaptive/2(x)
  Mux16/1 -> To Workspace9/1
  Pulse Generator11/1 -> Add13/1
  Ref Theta8/1 -> Add13/2
  Add13/1 -> [scl_x_ref], To Workspace10/1  "Reference"
  [scl_x_ref] -> Scope18/1
  Mux17/1 -> To Workspace4/1
  Mux7/1 -> To Workspace5/1
  From9/1 -> STW SMC/3(f(x))
  From12/1 -> STW SMC/5(x_ref)
  From11/1 -> STW SMC/4(g(x))
  From10/1 -> STW SMC/2(x)
  MPC Controller/1 -> Mux18/1, Scope4/1, Subsystem12/2(u (N))
  Subsystem12/1(Pos_1) -> Mux18/2, Mux8/1  "x1"
  Subsystem12/2(Pos_2) -> Mux18/3, Mux8/2, Scope3/1  "x2"
  Subsystem12/3(Vel_1) -> Mux18/4, Mux8/3  "v1"
  Subsystem12/4(Vel_2) -> Mux18/5, Scope21/1, Mux8/4  "v2"
  Mux8/1 -> MPC Controller/1
  [x_ref] -> MPC Controller/2
  [scl_x_ref] -> Scope3/2
  Band-Limited White Noise11/1 -> Subsystem12/1(disturbance)
  Mux18/1 -> To Workspace11/1
  Band-Limited White Noise12/1 -> Subsystem13/1(disturbance)
  Subsystem13/1(Pos_1) -> Mux19/1, Goto9/1  "x1"
  Subsystem13/2(Pos_2) -> Mux19/2, Add14/1, Goto10/1  "x2"
  Subsystem13/3(Vel_1) -> Mux19/3  "v1"
  Subsystem13/4(Vel_2) -> Mux19/4  "v2"
  From15/1 -> Mux19/5, Add14/2
  Add14/1 -> Goto5/1, Mux19/6
  IsDone/1(is_done) -> Goto8/1
  IsDone/5(next_ref_prev) -> Unit Delay3/1
  IsDone/4(next_step_size) -> Unit Delay2/1
  IsDone/3(next_time_since_change) -> Reward/4(time_since_change), Unit Delay1/1
  IsDone/2(next_timer_03) -> Unit Delay/1
  Unit Delay3/1 -> IsDone/7(x2_ref_prev)
  Unit Delay2/1 -> IsDone/6(current_step_size)
  Unit Delay1/1 -> IsDone/5(time_since_change)
  Unit Delay/1 -> IsDone/4(timer_03)
  From18/1 -> IsDone/1(x1)
  From19/1 -> IsDone/2(x2)
  From20/1 -> IsDone/3(x2_ref)
  Reward/1(reward) -> Goto7/1
  Reward/2(next_x2_prev) -> Unit Delay4/1
  From17/1 -> Reward/3(u)
  Unit Delay4/1 -> Reward/5(x2_prev)
  From21/1 -> Reward/1(x2)
  From22/1 -> Reward/2(x2_ref)
  From23/1 -> RL Agent/3
  From24/1 -> RL Agent/2
  Mux19/1 -> RL Agent/1
  RL Agent/1 -> Rate Limiter/1
  Rate Limiter/1 -> Subsystem13/2(u (N))
  Saturation9/1 -> Add15/1, Unit Delay5/1, Rate Transition/1
  MinMax Running Resettable1/1 -> Display2/1
  MinMax Running Resettable/1 -> Display3/1
  Add15/1 -> Display4/1, MinMax Running Resettable1/1, MinMax Running Resettable/1
  Unit Delay5/1 -> Add15/2
  Rate Limiter3/1 -> Saturation9/1
  Uniform Random Number/1 -> Rate Limiter3/1  "Reference"
  Rate Transition/1 -> Scope24/1
  Rate Transition2/1 -> Scope26/1
  Uniform Random Number2/1 -> Rate Limiter4/1  "Reference"
  Rate Limiter4/1 -> Saturation11/1
  Saturation11/1 -> Rate Transition2/1
  Rate Transition1/1 -> MinMax Running Resettable3/1, MinMax Running Resettable2/1, Mean/1
  Mean/1 -> Display5/1
  MinMax Running Resettable3/1 -> Display7/1
  MinMax Running Resettable2/1 -> Display6/1
  Sum18/1 -> Assignment1/2
  Saturation10/1 -> Mux20/1, Subsystem14/1(u)
  Sum21/1 -> Saturation10/1
  PID_Theta/1 -> Sum21/1
  PID_Pos/1 -> Sum21/2
  Band-Limited White Noise13/1 -> Sum21/3
  Subsystem14/4(pos_dot) -> Mux20/5  "x dot"
  Subsystem14/3(pos) -> Mux20/4, Scope27/2, Sum20/2  "Position"
  Subsystem14/2(theta_dot) -> Mux20/3  "Thetha dot"
  Subsystem14/1(theta) -> Mux20/2, Sum19/2, Scope25/2  "Theta"
  Mux20/1 -> To Workspace12/1
  Sum20/1 -> PID_Pos/1
  Ref Theta9/1 -> [IP_Theta_ref], Sum19/1
  Sum19/1 -> PID_Theta/1
  Ref position3/1 -> [IP_Pos_ref], Sum20/1
  [IP_Theta_ref] -> Scope25/1
  [IP_Pos_ref] -> Scope27/1
  PID_Theta1/1 -> Sum24/1
  Sum24/1 -> Saturation12/1
  Sum22/1 -> PID_Theta1/1
  Add16/1 -> Rate Limiter5/1
  Mux21/1 -> To Workspace13/1
  Sum23/1 -> PID_Pos1/1
  Subsystem15/1(theta) -> Mux21/2, Sum22/2, Scope28/2  "Theta"
  Ref Theta10/1 -> Sum22/1
  Subsystem15/2(theta_dot) -> Mux21/3  "Thetha dot"
  Band-Limited White Noise14/1 -> Sum24/3
  Subsystem15/4(pos_dot) -> Mux21/5  "x dot"
  PID_Pos1/1 -> Sum24/2
  Subsystem15/3(pos) -> Mux21/4, Scope29/2, Sum23/2  "Position"
  Ref Theta11/1 -> Add16/2
  Pulse Generator12/1 -> Add16/1
  Subsystem16/4(pos_dot) -> Mux23/4, Mux22/5  "x dot"
  Subsystem16/3(pos) -> Mux22/4, Mux23/3, Scope32/2  "Position"
  Subsystem16/2(theta_dot) -> Mux23/2, Mux22/3  "Thetha dot"
  Subsystem16/1(theta) -> Mux23/1, Scope31/2, Mux22/2  "Theta"
  Reshape3/1 -> Sliding Mode Controller (Reaching Law)4/1, MatrixMultiply4/2
  Mux23/1 -> Reshape3/1
  Saturation12/1 -> Scope30/1, Mux21/1, Subsystem15/1(u)
  Saturation13/1 -> Scope33/1, Mux22/1, Subsystem16/1(u)
  MatrixMultiply4/1 -> Sliding Mode Controller (Reaching Law)4/2
  A_4/1 -> MatrixMultiply4/1
  B4/1 -> Sliding Mode Controller (Reaching Law)4/3
  Sliding Mode Controller (Reaching Law)4/1 -> Sum25/1
  Sum25/1 -> Saturation13/1
  Band-Limited White Noise15/1 -> Sum25/2
  Constant2/1 -> Assignment2/1
  Add18/1 -> To Workspace14/1, [ip_ref], Assignment2/2  "Reference"
  Ref Theta14/1 -> Add18/2
  Pulse Generator14/1 -> Add18/1
  Assignment2/1 -> Rate Limiter2/1  "Reference"
  Rate Limiter2/1 -> Sliding Mode Controller (Reaching Law)4/4
  Rate Limiter5/1 -> Sum23/1
  Constant3/1 -> Scope31/1
  [ip_ref] -> Scope32/1
  Zero/1 -> Scope28/1
  [ip_ref] -> Scope29/1
  Mux22/1 -> To Workspace15/1
